simulink library "lib_TerCtrl_Scheduled"  (R2026a)
settings: Solver=VariableStepAuto
undefined symbols (not defined in the file): buses_lf, Psche, Qs_lf, vs_lf
settings Model: Creator=atomas  LastModifiedBy=atomas

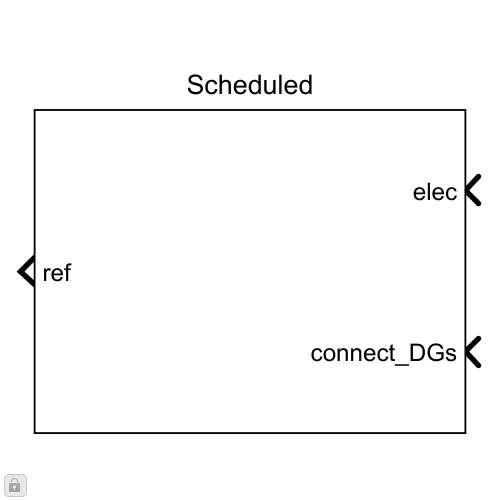
[thumbnail: Simulink's stored preview of the top-level diagram]
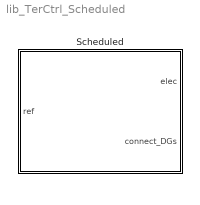
== system lib_TerCtrl_Scheduled ==
  Scheduled : Subsystem  VariantControl=Scheduled

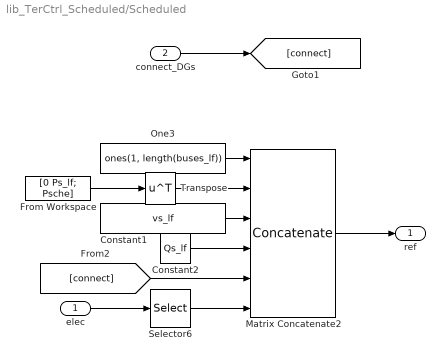
== system lib_TerCtrl_Scheduled/Scheduled ==
  elec : Inport
  connect_DGs : Inport  Port=2
  Constant1 : Constant  Value=vs_lf  VectorParams1D=off
  Constant2 : Constant  Value=Qs_lf  VectorParams1D=off
  From Workspace : FromWorkspace  VariableName=[0 Ps_lf; Psche]  SampleTime=Psche(1,1)  Interpolate=off  OutputAfterFinalValue=Holding final value
  Matrix Concatenate2 : Concatenate  NumInputs=6  Mode=Multidimensional array
  One3 : Constant  Value=ones(1, length(buses_lf))  VectorParams1D=off  OutDataTypeStr=Inherit: Inherit via back propagation
  Selector6 : Selector  NumberOfDimensions=2  InputPortWidth=3  IndexOptions=Index vector (dialog),Select all  Indices=6,1  OutputSizes=1,1
  Transpose : Math  Operator=transpose
  ref : Outport
  wires:
  Transpose/1 -> Matrix Concatenate2/2
  From Workspace/1 -> Transpose/1
  Constant2/1 -> Matrix Concatenate2/4
  Constant1/1 -> Matrix Concatenate2/3
  One3/1 -> Matrix Concatenate2/1
  [connect] -> Matrix Concatenate2/5
  Selector6/1 -> Matrix Concatenate2/6
  Matrix Concatenate2/1 -> ref/1
  connect_DGs/1 -> [connect]
  elec/1 -> Selector6/1
